simulink model "Simulink_simulation"  (R2025b)
settings: Solver=VariableStepAuto  StartTime=0.0  StopTime=30  RelTol=1e-3
libraries: SignalEditorBlockLib x2, sim3dlib x1, uavsim3dlib x1
settings Model: Creator=amirs  LastModifiedBy=amirs

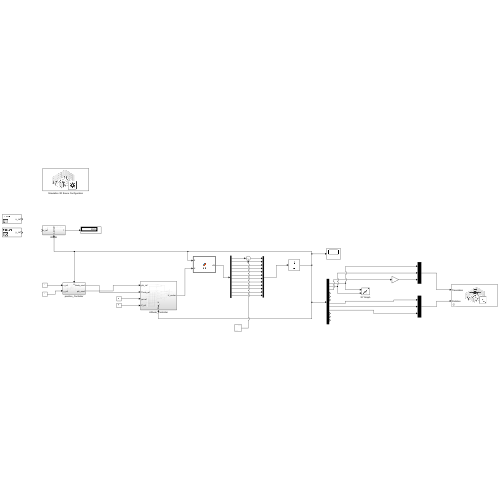
[thumbnail: Simulink's stored preview of the top-level diagram]
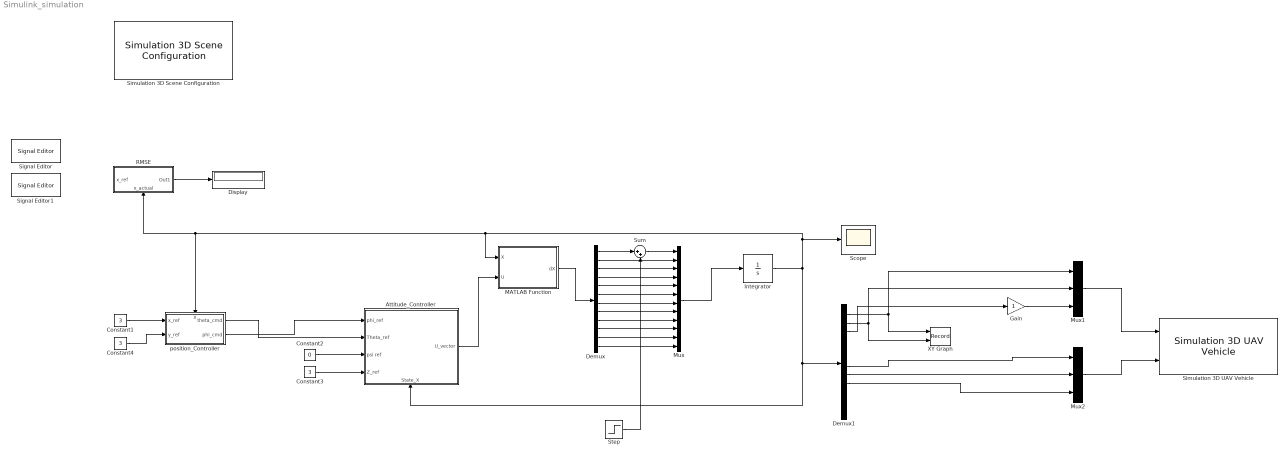
== system Simulink_simulation ==
  Attitude_Controller : Subsystem
      settings: PortSchema="{\"entries\":[{\"content\":{\"sides\":[{\"content\":{\"connectorIds\":[\"In1\",\"In2\",\"In3\",\"In4\"]},\"type\":\"ConnectorPlacement.EquallySpacedRectSide\",\"uuid\":\"19f4eeea-d5cb-4ed7-9c59-67184399f9de\"},{\"content\":{\"connectorIds\":[\"Out1\"],\"side\":\"RIGHT\"},\"type\":\"ConnectorPlacement.EquallySpacedRectSide\",\"uuid\":\"b3f5ec5c-a38f-4295-9bcf-0fae3bfa674b\"},{\"content\":{\"side\":\"TOP\"},\"type\":\"ConnectorPlacement.EquallySpacedRectSide\",\"uuid\":\"2fc47e81-4ab5-4bbe-b029-56bfdcdb6174\"},{\"content\":{\"connectorIds\":[\"In5\"],\"side\":\"BOTTOM\"},\"type\":\"ConnectorPlacement.EquallySpacedRectSide\",\"uuid\":\"a7c3fd73-d82a-467d-bca9-1f7d01263d9c\"}]},\"type\":\"ConnectorPlacement.EquallySpacedConnector\",\"uuid\":\"700c1ad5-606a-4180-bf9f-c597a2a2a5d4\"}],\"packageUris\":[\"http://schema.mathworks.com/mf0/Connector/R2020b\"],\"version\":\"1.0\"}"
  Constant1 : Constant  Value=3
  Constant2 : Constant  Value=0
  Constant3 : Constant  Value=3
  Constant4 : Constant  Value=3
  Demux : Demux  Outputs=12
  Demux1 : Demux  Outputs=12
  Display : Display
  Gain : Gain
  Integrator : Integrator  InitialCondition=[0;0;0;0;0;0;0;0;0;0;0;0]
  MATLAB Function : MATLAB Function  TreatAsAtomicUnit=on
  Mux : Mux  Inputs=12
  Mux1 : Mux  Inputs=3
  Mux2 : Mux  Inputs=3
  RMSE : Subsystem
      settings: PortSchema="{\"entries\":[{\"content\":{\"sides\":[{\"content\":{\"connectorIds\":[\"In1\"]},\"type\":\"ConnectorPlacement.EquallySpacedRectSide\",\"uuid\":\"5e07c89f-ef09-4b0a-bed5-e0d03eb8d545\"},{\"content\":{\"connectorIds\":[\"Out1\"],\"side\":\"RIGHT\"},\"type\":\"ConnectorPlacement.EquallySpacedRectSide\",\"uuid\":\"9156e923-85eb-42fc-9dec-5f08a3c9d42c\"},{\"content\":{\"side\":\"TOP\"},\"type\":\"ConnectorPlacement.EquallySpacedRectSide\",\"uuid\":\"e2ee007b-856b-4d03-8afd-b743321baf7d\"},{\"content\":{\"connectorIds\":[\"In2\"],\"side\":\"BOTTOM\"},\"type\":\"ConnectorPlacement.EquallySpacedRectSide\",\"uuid\":\"3aca7e9a-13ba-49c1-8015-1f7d41362bc4\"}]},\"type\":\"ConnectorPlacement.EquallySpacedConnector\",\"uuid\":\"905e6a99-45d0-4759-a1dd-bed499fabe76\"}],\"packageUris\":[\"http://schema.mathworks.com/mf0/Connector/R2020b\"],\"version\":\"1.0\"}"
  Scope : Scope
      settings: ActiveDisplayYMinimum=-6.4871029575674033  ActiveDisplayYMaximum=8.1253486671858823
  Signal Editor : SignalEditorBlockLib/Signal Editor  FileName=squer.mat  ActiveScenario=Scenario  ActiveSignal=x_ref  IsBus=off  OutputBusObjectStr=Bus: BusObject  SampleTime=0  ZeroCross=off  OutputAfterFinalValue=Setting to zero  Unit=inherit  PreserveSignalName=on  ApplySigPropsToAllScenarios=on  ApplySigPropsToAllSignals=off  SignalPropertySource=Dialog parameters
  Signal Editor1 : SignalEditorBlockLib/Signal Editor  FileName=squer_y.mat  ActiveScenario=Scenario  ActiveSignal=y_ref  IsBus=off  OutputBusObjectStr=Bus: BusObject  SampleTime=0  ZeroCross=off  OutputAfterFinalValue=Setting to zero  Unit=inherit  PreserveSignalName=on  ApplySigPropsToAllScenarios=on  ApplySigPropsToAllSignals=off  SignalPropertySource=Dialog parameters
  Simulation 3D Scene Configuration : sim3dlib/Simulation 3D Scene Configuration  Priority=0  ProjectFormat=Default Scenes  SceneDesc=US city block  ProjectName=C:\Program Files\MATLAB\R2025b\toolbox\shared\sim3d_projects\automotive_project_windows\UE\WindowsNoEditor\VehicleSimulation.exe  ScenePath=/Game/Maps/USCityBlock  EnableOpenDRIVE=off  vehTagList={'Custom';'Scene Origin';'SimulinkVehicle1'}  vehTag=Scene Origin  AttachedCameraRelativeTranslation=[0 0 0]  FreeCameraDefaultInitialTranslation=[-6, 0, 2]  AttachedCameraRelativeRotation=[0 0 0]  FreeCameraDefaultInitialRotation=[0, -15, 0]  ViewpointName=Custom  FreeCameraInitialTranslation=[0, 0, 0]  ViewpointTranslation=[0, 0, 0]  FreeCameraInitialRotation=[0, 0, 0]  ViewpointRotation=[0, 0, 0]  OpVisEn=off  Ts=1/60  EnableWindow=on  EnableRemoteAccess=off  EnableWeather=off  SunAzimuth=90  SunAltitude=40.0  EnableGeospatialSun=off  Latitude=0  Longitude=0  Date=2023-01-01  Time=10:30:00  GeoTimeZone=-5.0  SunDaylightSaving=off  wind=1  clouds=10  EnableVolumetricClouds=off  CloudCoverage=0  CloudAltitude=6  fog=0  rain=0  RaindropsEffect=off  SnowDensity=0  EnableGeospatial=off  TilesetSource=Earth terrain  UseTrueOrigin=off  OriginHeight=200  OriginLatitude=40.744652  OriginLongitude=-73.988864  MapStyle=Aerial  AdditionalAssetIDs=[]  UseAdvancedSunSky=off  SolarTime=11  TimeZone=-5  Day=21  Month=9  Year=2022  UseDaylightSavingTime=on  DSTStartDay=10  DSTStartMonth=3  DSTEndDay=3  DSTEndMonth=11  DSTSwitchHour=2  sensorTag=MainCamera1  sensorId=1  sensorName=MainCamera1  mountLoc=Origin  offsetFlag=off  tmountOffset=[0, 0, 0]  rmountOffset=[0, 0, 0]  HorizontalResolution=1280  VerticalResolution=720  HorizontalFOV=60  mountPoint=[0 0 0]  mountOrientation=[0 0 0]  aMode=4  ID=1  GeoTrigger=Inactive  ViewNameList={'Custom'}  ViewTranslationList={'[0 0 0]'}  ViewRotationList={'[0 0 0]'}
      settings: LibrarySourceBlock=uavsim3dlib/Simulation 3D Scene Configuration
  Simulation 3D UAV Vehicle : uavsim3dlib/Simulation 3D UAV Vehicle  Priority=-1  Mesh=Quadrotor  MeshPath=/MathWorksUAVContent/UAVs/HexaRotorUAV/HexaRotor.HexaRotor  Color=Green  ActorName=SimulinkVehicle1  UseGlobalFrame=off  InitialTranslation=[0 0 0]  InitialRotation=[0 0 0]  InitialTranslationGlobal=[0 0 0]  InitialGeoOrigin=[0 0 0]  InitialRotationGlobal=[0 0 0]  SampleTime=-1  ActorType=SimulinkVehicle  ID=1  aMode=4  ActorTag=SimulinkVehicle1
  Step : Step  Time=25  After=0  SampleTime=0
  Sum : Sum  Inputs=|++
  XY Graph : Record  NumPorts=2.0  FileSettingsInternal="{\"entries\":[{\"content\":{\"excelSettings\":{\"content\":{},\"type\":\"Streamout.ExcelSettings\"},\"parquetSettings\":{\"content\":{},\"type\":\"Streamout.ParquetSettings\"}},\"type\":\"Streamout.FileSettingStorage\",\"uuid\":\"\"}],\"packageUris\":[\"http:\\/\\/schema.mathworks.com\\/mf0\\/streamout_blocks\\/R2020a\"],\"version\":\"1.0\"}"  FrameSettings=[0, 0]  Layout=[1 1]  SignalsInternal="{\"entries\":[{\"content\":{\"signals\":[{\"content\":{\"blockPath\":[],\"dimensions\":[1],\"domain\":\"\",\"lineColor\":\"#a2142f\",\"plots\":[ 1 ],\"port\":1,\"sid\":[\"\"],\"signalID\":1,\"signalName\":\"Demux1:1\"},\"type\":\"RecordBlkView.Signal\",\"uuid\":\"\"},{\"content\":{\"blockPath\":[],\"dimensions\":[1],\"domain\":\"\",\"lineColor\":\"#139fff\",\"plots\":[ 1 ],\"port\":2,\"sid\":[\"\"],\"signalID\":2,\"signalName\":\"Demux1:2\"},\"type\":\"RecordBlkView.Signal\",\"uuid\":\"\"}]},\"type\":\"RecordBlkView.InputSignals\",\"uuid\":\"\"}],\"packageUris\":[\"http:\\/\\/schema.mathworks.com\\/mf0\\/streamout_blocks\\/R2020a\"],\"version\":\"1.0\"}"  VisualizationBindings="{\"xyplotplugin\":{\"info\":[{\"series\":[{\"bindingParametersList\":[{\"parameter\":\"X-Axis\",\"signalID\":1,\"signalName\":\"Demux1:1\"},{\"parameter\":\"Y-Axis\",\"signalID\":2,\"signalName\":\"Demux1:2\"}],\"seriesID\":0}],\"subplotID\":1}]}}"  CompatibilityTag=XY
  position_Controller : Subsystem
      settings: PortSchema="{\"entries\":[{\"content\":{\"sides\":[{\"content\":{\"connectorIds\":[\"In1\",\"In2\"]},\"type\":\"ConnectorPlacement.EquallySpacedRectSide\",\"uuid\":\"b3fdc6c0-3d6b-4fed-ba04-72ee8971ce33\"},{\"content\":{\"connectorIds\":[\"Out1\",\"Out2\"],\"side\":\"RIGHT\"},\"type\":\"ConnectorPlacement.EquallySpacedRectSide\",\"uuid\":\"c5fff90f-3f0d-4e66-bfd3-42639056edf5\"},{\"content\":{\"connectorIds\":[\"In3\"],\"side\":\"TOP\"},\"type\":\"ConnectorPlacement.EquallySpacedRectSide\",\"uuid\":\"29c618c7-b581-4d0e-90c8-5996712070e8\"}]},\"type\":\"ConnectorPlacement.EquallySpacedConnector\",\"uuid\":\"86696893-c9ee-41ff-bf75-cf6f558ac07e\"}],\"packageUris\":[\"http://schema.mathworks.com/mf0/Connector/R2020b\"],\"version\":\"1.0\"}"
  wires:
  Integrator/1 -> Scope/1, MATLAB Function/1(X), RMSE/2(x_actual), position_Controller/3(X), Demux1/1, Attitude_Controller/5(State_X)
  Constant2/1 -> Attitude_Controller/3(psi ref)
  Constant3/1 -> Attitude_Controller/4(Z_ref)
  position_Controller/2(phi_cmd) -> Attitude_Controller/1(phi_ref)
  position_Controller/1(theta_cmd) -> Attitude_Controller/2(Theta_ref)
  Attitude_Controller/1(U_vector) -> MATLAB Function/2(U)
  Step/1 -> Sum/2
  Demux/1 -> Sum/1
  Sum/1 -> Mux/1
  Demux/2 -> Mux/2
  Demux/3 -> Mux/3
  Demux/4 -> Mux/4
  Demux/5 -> Mux/5
  Demux/6 -> Mux/6
  Demux/7 -> Mux/7
  Demux/8 -> Mux/8
  Demux/9 -> Mux/9
  Demux/10 -> Mux/10
  Demux/11 -> Mux/11
  Demux/12 -> Mux/12
  MATLAB Function/1(dX) -> Demux/1
  Mux/1 -> Integrator/1
  RMSE/1(Out1) -> Display/1
  Demux1/1 -> Mux1/1, XY Graph/1
  Demux1/2 -> XY Graph/2, Mux1/2
  Demux1/3 -> Gain/1
  Gain/1 -> Mux1/3
  Mux1/1 -> Simulation 3D UAV Vehicle/1
  Demux1/7 -> Mux2/1
  Demux1/8 -> Mux2/2
  Demux1/9 -> Mux2/3
  Mux2/1 -> Simulation 3D UAV Vehicle/2
  Constant1/1 -> position_Controller/1(x_ref)
  Constant4/1 -> position_Controller/2(y_ref)

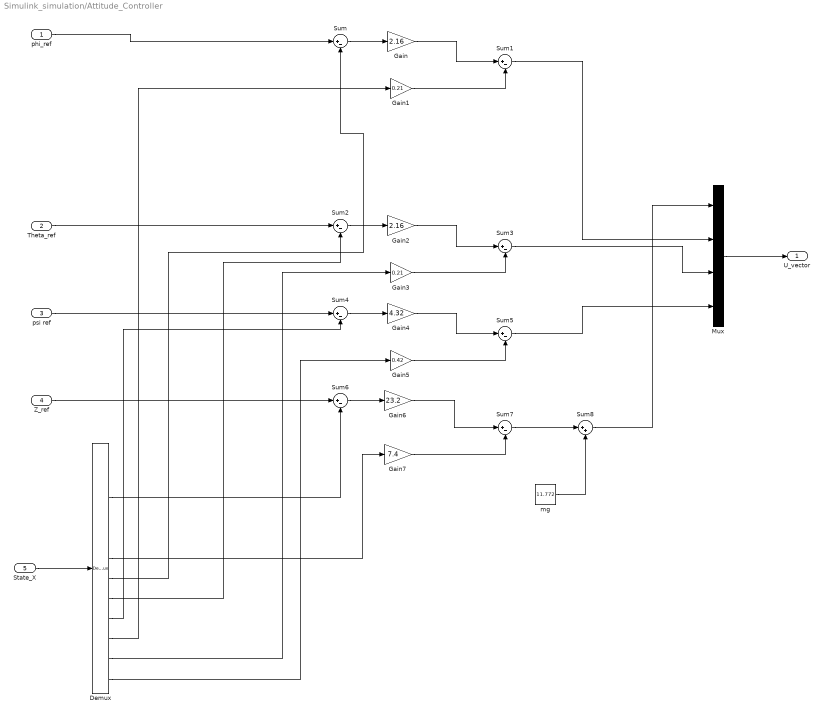
== system Simulink_simulation/Attitude_Controller ==
  phi_ref : Inport
  Theta_ref : Inport  Port=2
  psi ref : Inport  Port=3
  Z_ref : Inport  Port=4
  State_X : Inport  Port=5
  Demux : Demux  Outputs=12
  Gain : Gain  Gain=2.16
  Gain1 : Gain  Gain=0.21
  Gain2 : Gain  Gain=2.16
  Gain3 : Gain  Gain=0.21
  Gain4 : Gain  Gain=4.32
  Gain5 : Gain  Gain=0.42
  Gain6 : Gain  Gain=23.2
  Gain7 : Gain  Gain=7.4
  Mux : Mux
  Sum{,1..7} (8 alike) : Sum  Inputs=|+-
  Sum8 : Sum  Inputs=|++
  mg : Constant  Value=11.772
  U_vector : Outport
  wires:
  State_X/1 -> Demux/1
  phi_ref/1 -> Sum/1
  Demux/7 -> Sum/2
  Sum/1 -> Gain/1
  Demux/10 -> Gain1/1
  Gain/1 -> Sum1/1
  Gain1/1 -> Sum1/2
  Gain3/1 -> Sum3/2
  Gain2/1 -> Sum3/1
  Sum2/1 -> Gain2/1
  Theta_ref/1 -> Sum2/1
  Demux/8 -> Sum2/2
  Demux/11 -> Gain3/1
  Gain5/1 -> Sum5/2
  Gain4/1 -> Sum5/1
  Sum4/1 -> Gain4/1
  psi ref/1 -> Sum4/1
  Demux/9 -> Sum4/2
  Demux/12 -> Gain5/1
  Z_ref/1 -> Sum6/1
  Demux/3 -> Sum6/2
  Sum6/1 -> Gain6/1
  Demux/6 -> Gain7/1
  Gain6/1 -> Sum7/1
  Gain7/1 -> Sum7/2
  Sum7/1 -> Sum8/1
  mg/1 -> Sum8/2
  Sum8/1 -> Mux/1
  Sum1/1 -> Mux/2
  Sum3/1 -> Mux/3
  Sum5/1 -> Mux/4
  Mux/1 -> U_vector/1

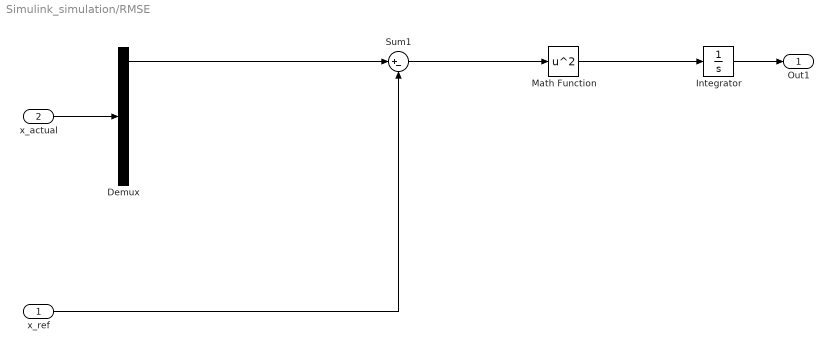
== system Simulink_simulation/RMSE ==
  x_ref : Inport
  x_actual : Inport  Port=2
  Demux : Demux  Outputs=12
  Integrator : Integrator
  Math Function : Math  Operator=square
  Sum1 : Sum  Inputs=|+-
  Out1 : Outport
  wires:
  x_actual/1 -> Demux/1
  x_ref/1 -> Sum1/2
  Demux/1 -> Sum1/1
  Sum1/1 -> Math Function/1
  Math Function/1 -> Integrator/1
  Integrator/1 -> Out1/1

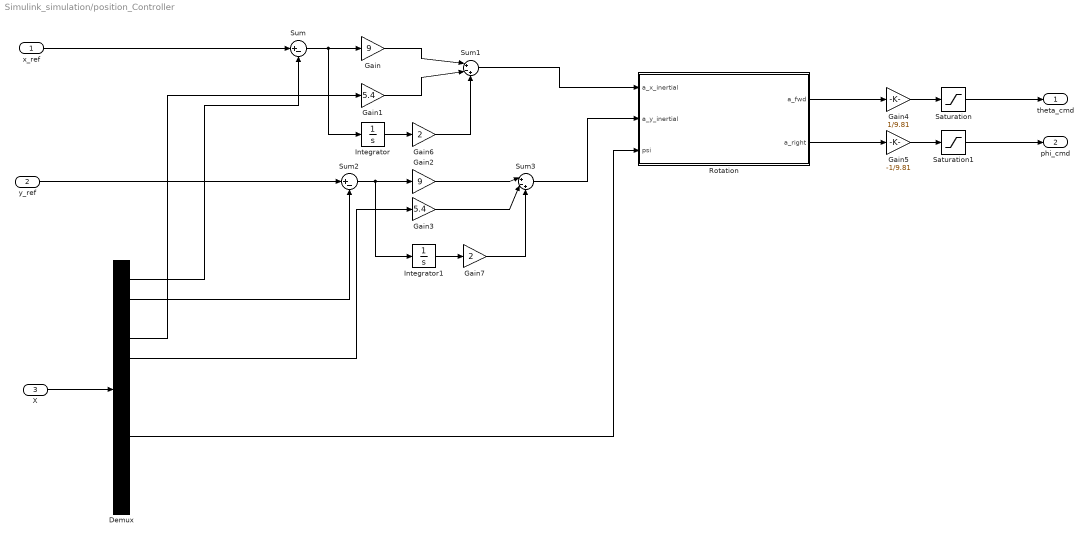
== system Simulink_simulation/position_Controller ==
  x_ref : Inport
  y_ref : Inport  Port=2
  X : Inport  Port=3
  Demux : Demux  Outputs=12
  Gain : Gain  Gain=9
  Gain1 : Gain  Gain=5.4
  Gain2 : Gain  Gain=9
  Gain3 : Gain  Gain=5.4
  Gain4 : Gain  Gain=1/9.81
  Gain5 : Gain  Gain=-1/9.81
  Gain6 : Gain  Gain=2
  Gain7 : Gain  Gain=2
  Integrator : Integrator  LimitOutput=on  UpperSaturationLimit=5  LowerSaturationLimit=-5
  Integrator1 : Integrator  LimitOutput=on  UpperSaturationLimit=5  LowerSaturationLimit=-5
  Rotation : Subsystem
  Saturation : Saturate  UpperLimit=0.2  LowerLimit=-0.2
  Saturation1 : Saturate  UpperLimit=0.2  LowerLimit=-0.2
  Sum : Sum  Inputs=|+-
  Sum1 : Sum  Inputs=|+-+
  Sum2 : Sum  Inputs=|+-
  Sum3 : Sum  Inputs=|+-+
  theta_cmd : Outport
  phi_cmd : Outport  Port=2
  wires:
  X/1 -> Demux/1
  x_ref/1 -> Sum/1
  Demux/1 -> Sum/2
  Sum/1 -> Integrator/1, Gain/1
  Demux/4 -> Gain1/1
  Gain/1 -> Sum1/1
  Gain1/1 -> Sum1/2
  Gain3/1 -> Sum3/2
  Gain2/1 -> Sum3/1
  Sum2/1 -> Integrator1/1, Gain2/1
  y_ref/1 -> Sum2/1
  Demux/2 -> Sum2/2
  Demux/5 -> Gain3/1
  Sum3/1 -> Rotation/2(a_y_inertial)
  Demux/9 -> Rotation/3(psi)
  Rotation/1(a_fwd) -> Gain4/1
  Gain4/1 -> Saturation/1
  Saturation/1 -> theta_cmd/1
  Rotation/2(a_right) -> Gain5/1
  Gain5/1 -> Saturation1/1
  Saturation1/1 -> phi_cmd/1
  Sum1/1 -> Rotation/1(a_x_inertial)
  Integrator/1 -> Gain6/1
  Gain6/1 -> Sum1/3
  Integrator1/1 -> Gain7/1
  Gain7/1 -> Sum3/3

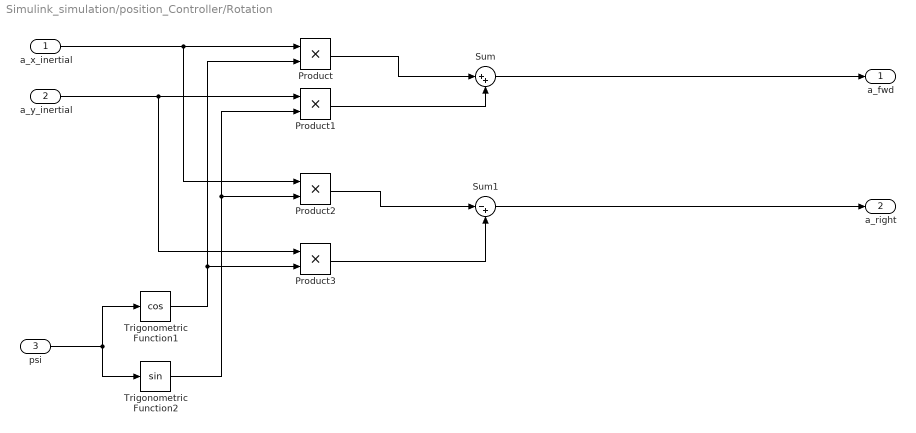
== system Simulink_simulation/position_Controller/Rotation ==
  a_x_inertial : Inport
  a_y_inertial : Inport  Port=2
  psi : Inport  Port=3
  Product{,1..3} (4 alike) : Product
  Sum : Sum  Inputs=|++
  Sum1 : Sum  Inputs=|-+
  Trigonometric Function1 : Trigonometry  Operator=cos
  Trigonometric Function2 : Trigonometry
  a_fwd : Outport
  a_right : Outport  Port=2
  wires:
  psi/1 -> Trigonometric Function2/1, Trigonometric Function1/1
  a_x_inertial/1 -> Product2/1, Product/1
  Trigonometric Function1/1 -> Product3/2, Product/2
  a_y_inertial/1 -> Product3/1, Product1/1
  Trigonometric Function2/1 -> Product2/2, Product1/2
  Product/1 -> Sum/1
  Product1/1 -> Sum/2
  Sum/1 -> a_fwd/1
  Product2/1 -> Sum1/1
  Product3/1 -> Sum1/2
  Sum1/1 -> a_right/1

== matlab function Simulink_simulation/MATLAB Function ==
  data: X input; dX output; U input
function dX=fcn(X,U)
        m= 1.2;
        g=9.81;
        Ixx=0.01;Iyy=0.01;Izz=0.02;
        phi=X(7);theta=X(8);psi=X(9);
        p = X(10);q=X(11);r=X(12);
        U1=U(1);U2=U(2);U3=U(3);U4=U(4);

        % Rotational Dyanamics:
        p_dot = (U2-(Izz-Iyy)*q*r)/Ixx;
        q_dot = (U3-(Ixx-Izz)*p*r)/Iyy;
        r_dot = (U4-(Iyy-Ixx)*p*q)/Izz;

        % 
        phi_dot= p + q*sin(phi)*tan(theta) + r*cos(phi)*tan(theta);
        theta_dot = q*cos(phi)-r*sin(phi);
        psi_dot = q*sin(phi)/cos(theta) + r*cos(phi)/cos(theta);

        % Translational
        ax = (U1/m)*(cos(phi)*sin(theta)*cos(psi) + sin(phi)*sin(psi));
        ay = (U1/m)*(cos(phi)*sin(theta)*sin(psi)- sin(phi)*cos(psi));
        az = (-1*g) + (U1/m)*(cos(phi)*cos(theta));

        dX = [X(4);X(5);X(6);ax;ay;az;phi_dot;theta_dot;psi_dot;p_dot;q_dot;r_dot];
end
